simulink model "odst_transfer_sim"  (R2026b)
settings: Solver=ode45  StartTime=-odst_burnplan.tau  StopTime=odst_tstop  MaxStep=odst_burnplan.tau/4  RelTol=1e-9  AbsTol=1e-9
undefined symbols (not defined in the file or in its folder): odst_sim_dynamics, odst_x0
settings Model: LastModifiedBy=thedh

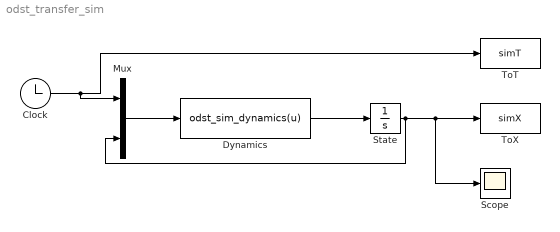
== system odst_transfer_sim ==
  Clock : Clock
  Dynamics : MATLABFcn  MATLABFcn=odst_sim_dynamics(u)  OutputDimensions=6
  Mux : Mux  Inputs=2
  Scope : Scope
  State : Integrator  InitialCondition=odst_x0
  ToT : ToWorkspace  VariableName=simT  SampleTime=-1
  ToX : ToWorkspace  VariableName=simX  SampleTime=-1
  wires:
  Clock/1 -> Mux/1, ToT/1
  State/1 -> ToX/1, Scope/1, Mux/2
  Mux/1 -> Dynamics/1
  Dynamics/1 -> State/1
